simulink model "gm_uz_resolver_multiturn"  (R2025a)
settings: Solver=FixedStepDiscrete  StartTime=0.0  StopTime=2  RelTol=1e-3
settings Model: Creator=jonat  LastModifiedBy=jonat
settings SolverCC: AlgebraicLoopSolver=TrustRegion
settings DataIOCC: LimitDataPoints=on  SaveOutput=off  SaveTime=off
settings OptimizationCC: BlockReduction=off  ConditionallyExecuteInputs=off  DefaultParameterBehavior=Inlined  InheritOutputTypeSmallerThanSingle=on  LifeSpan=inf
settings DebuggingCC: AlgebraicLoopMsg=error  InheritedTsInSrcMsg=none  SingleTaskRateTransMsg=error  UnconnectedInputMsg=warning  UnconnectedOutputMsg=warning  UnconnectedLineMsg=warning  AllowSymbolicDim=off  StrictBusMsg=ErrorOnBusTreatedAsVector  SFUnexpectedBacktrackingDiag=warning  SFNoUnconditionalDefaultTransitionDiag=warning  SFExecutionAtInitializationDiag=none  ArithmeticOperatorsInVariantConditions=warning
settings HardwareCC: ProdBitPerPointer=32.0  ProdBitPerSizeT=32.0  ProdBitPerPtrDiffT=32.0  ProdLargestAtomicFloat=None  ProdIntDivRoundTo=Undefined  ProdEndianess=Unspecified  ProdWordSize=32.0  ProdHWDeviceType=ASIC/FPGA->ASIC/FPGA  ProdEqTarget=off
settings ModelReferenceCC: EnableRefExpFcnMdlSchedulingChecks=on
settings SFSimCC: SimUseLocalCustomCode=off  CustomCodeUndefinedFunction=UseInterfaceOnly
settings RTWCC: RTWUseLocalCustomCode=off  GPUComputeCapability=3.5
settings CodeAppCC: StateflowObjectComments=on
settings GRTTargetCC: TargetLangStandard=C89/C90 (ANSI)
settings ConfigComp: CovScope=ReferencedModels  CovMetricSettings=dw  CovSaveCumulativeToWorkspaceVar=on  CovSaveSingleToWorkspaceVar=on  CovExternalEMLEnable=off  CovSFcnEnable=off

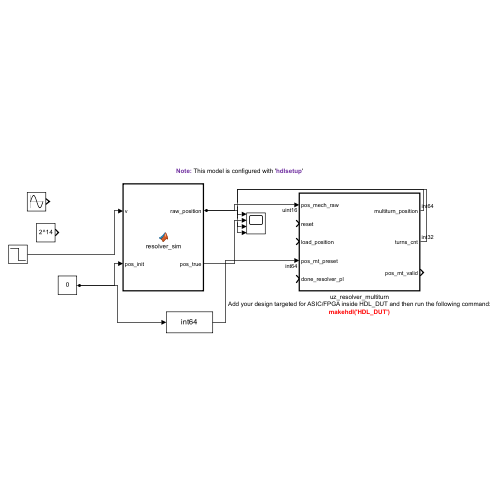
[thumbnail: Simulink's stored preview of the top-level diagram]
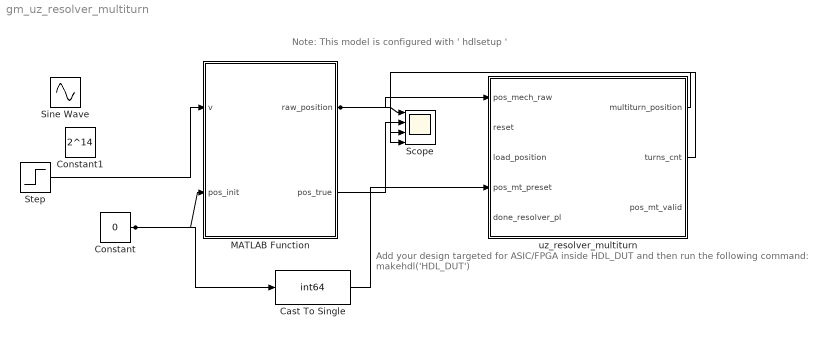
== system gm_uz_resolver_multiturn ==
  note: Add your design targeted for ASIC/FPGA inside HDL_DUT and then run the following command:
      | makehdl('HDL_DUT')
  note: Note: This model is configured with ' hdlsetup '
  Cast To Single : DataTypeConversion  OutDataTypeStr=int64  SaturateOnIntegerOverflow=off  RndMeth=Floor
  Constant : Constant  Value=0
  Constant1 : Constant  Value=2^14
  MATLAB Function : MATLAB Function  TreatAsAtomicUnit=on
  Scope : Scope  NumInputPorts=4
      settings: ActiveDisplayYMinimum=-46082.286781683193  ActiveDisplayYMaximum=89653.10837477204
  Sine Wave : Sin  Amplitude=20000  Frequency=2*pi  SampleTime=0
  Step : Step  Before=2^13  After=-2^13
  uz_resolver_multiturn : Subsystem  TreatAsAtomicUnit=on
  wires:
  uz_resolver_multiturn/2(turns_cnt) -> Scope/4
  Cast To Single/1 -> uz_resolver_multiturn/4(pos_mt_preset)
  uz_resolver_multiturn/1(multiturn_position) -> Scope/3
  MATLAB Function/2(pos_true) -> Scope/2
  MATLAB Function/1(raw_position) -> Scope/1, uz_resolver_multiturn/1(pos_mech_raw)
  Constant/1 -> Cast To Single/1, MATLAB Function/2(pos_init)
  Step/1 -> MATLAB Function/1(v)

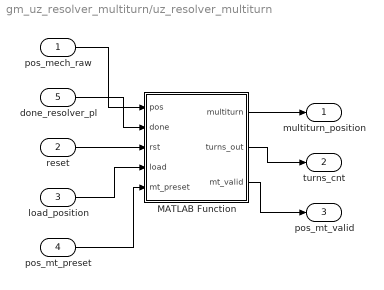
== system gm_uz_resolver_multiturn/uz_resolver_multiturn ==
  pos_mech_raw : Inport  OutDataTypeStr=uint16  PortDimensions=1  SampleTime=0.04
  reset : Inport  Port=2  OutDataTypeStr=boolean  PortDimensions=1  SampleTime=0.04
  load_position : Inport  Port=3  OutDataTypeStr=boolean  PortDimensions=1  SampleTime=0.04
  pos_mt_preset : Inport  Port=4  OutDataTypeStr=fixdt(1, 64, 0)  PortDimensions=1  SampleTime=0.04
  done_resolver_pl : Inport  Port=5  OutDataTypeStr=boolean  PortDimensions=1  SampleTime=0.04
  MATLAB Function : Subsystem
  multiturn_position : Outport  OutDataTypeStr=int64  SampleTime=0.04  VectorParamsAs1DForOutWhenUnconnected=off
  turns_cnt : Outport  Port=2  OutDataTypeStr=int32  SampleTime=0.04
  pos_mt_valid : Outport  Port=3  OutDataTypeStr=boolean  SampleTime=0.04
  wires:
  reset/1 -> MATLAB Function/3(rst)
  pos_mech_raw/1 -> MATLAB Function/1(pos)
  MATLAB Function/3(mt_valid) -> pos_mt_valid/1
  MATLAB Function/1(multiturn) -> multiturn_position/1
  done_resolver_pl/1 -> MATLAB Function/2(done)
  load_position/1 -> MATLAB Function/4(load)
  pos_mt_preset/1 -> MATLAB Function/5(mt_preset)
  MATLAB Function/2(turns_out) -> turns_cnt/1

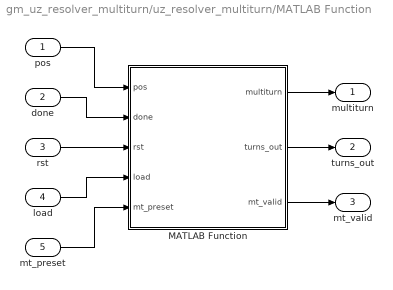
== system gm_uz_resolver_multiturn/uz_resolver_multiturn/MATLAB Function ==
  pos : Inport  OutDataTypeStr=uint16  PortDimensions=1  SampleTime=0.04
  done : Inport  Port=2  OutDataTypeStr=boolean  PortDimensions=1  SampleTime=0.04
  rst : Inport  Port=3  OutDataTypeStr=boolean  PortDimensions=1  SampleTime=0.04
  load : Inport  Port=4  OutDataTypeStr=boolean  PortDimensions=1  SampleTime=0.04
  mt_preset : Inport  Port=5  OutDataTypeStr=fixdt(1, 64, 0)  PortDimensions=1  SampleTime=0.04
  MATLAB Function : MATLAB Function  TreatAsAtomicUnit=on
  multiturn : Outport  SampleTime=0.04
  turns_out : Outport  Port=2  SampleTime=0.04
  mt_valid : Outport  Port=3  SampleTime=0.04
  wires:
  pos/1 -> MATLAB Function/1(pos)
  MATLAB Function/1(multiturn) -> multiturn/1
  done/1 -> MATLAB Function/2(done)
  rst/1 -> MATLAB Function/3(rst)
  load/1 -> MATLAB Function/4(load)
  MATLAB Function/3(mt_valid) -> mt_valid/1
  mt_preset/1 -> MATLAB Function/5(mt_preset)
  MATLAB Function/2(turns_out) -> turns_out/1

== matlab function gm_uz_resolver_multiturn/MATLAB Function ==
  data: v input; raw_position output; pos_init input; pos_true output
function [raw_position, pos_true] = resolver_sim(v, pos_init)
%RESOLVER_SIM  Simuliert einen Resolver als Signalquelle fuer multiturn_counter
%
%   Fuer einen MATLAB Function Block in Simulink (nur Testbench, nicht fuer HDL).
%
%   Eingaenge:
%     v             double   Geschwindigkeit in Counts pro Abtastschritt
%                            (65536 Counts = 1 Umdrehung, |v| < 32768 = 180 Grad)
%     pos_init      double   Startposition in Counts (wird nur im 1. Schritt gelesen)
%
%   Ausgaenge:
%     raw_position  uint16   Singleturn-Rohwert 0 ... 65535 (-> Eingang pos)
%     pos_true      int64    "Wahre" Multiturn-Position in Counts (Referenz)
%
%   Pruefung:
%     multiturn - pos_true muss zwischen zwei rst/load-Ereignissen konstant
%     und ein Vielfaches von 65536 sein. Bei richtig gesetztem mt_preset ist
%     die Differenz 0.

%#codegen

persistent p

if isempty(p)
    p = int64(round(pos_init));
end

% Ausgabe der aktuellen Position
pos_true     = p;
raw_position = uint16(mod(p, int64(65536)));

% Position fuer den naechsten Schritt weiterdrehen
p = p + int64(round(v));

end

== matlab function gm_uz_resolver_multiturn/uz_resolver_multiturn/MATLAB Function/MATLAB Function ==
  settings: fimath=fimath('RoundingMethod', 'Floor','OverflowAction', 'Wrap','ProductMode', 'FullPrecision', 'SumMode', 'FullPrecision')
  data: pos input; done input; multiturn output; rst input; load input; mt_preset input; turns_out output; mt_valid output
function [multiturn, turns_out, mt_valid] = multiturn_counter(pos, done, rst, load, mt_preset)
%MULTITURN_COUNTER  Multiturn-Zaehlung fuer Resolver-Singleturn (uint16)
%
%   Fuer den MATLAB Function Block in Simulink (HDL Coder tauglich).
%   Laeuft im FPGA-Systemtakt (z. B. 100 MHz). Gezaehlt wird nur bei der
%   steigenden Flanke von done (z. B. uz_resolver_pl_interface/done).
%   Funktioniert sowohl, wenn done ein Puls ist, als auch, wenn done ein
%   Pegel ist.
%
%   Eingaenge:
%     pos        uint16   Singleturn-Position (0 ... 65535), z. B. position_raw
%     done       boolean  Neuer, stabiler Positionswert liegt an
%     rst        boolean  Reset: turns = 0, naechster gueltiger Wert wird
%                         ohne Wrap-Pruefung als Startwert uebernommen
%     load       boolean  Letzte bekannte Multiturn-Position uebernehmen
%     mt_preset  int64    Gespeicherte Multiturn-Position (turns*65536 + pos)
%
%   Ausgaenge:
%     multiturn  int64    turns * 65536 + pos_last
%                         (untere 16 Bit = letzter gueltiger Singleturn-Rohwert)
%     turns_out  int32    Umdrehungszaehler
%     mt_valid   boolean  true, sobald multiturn einen gueltigen Bezug hat
%
%   Wrap-Erkennung ueber das Delta zwischen zwei gueltigen Werten:
%     delta < -32768  ->  Ueberlauf vorwaerts  (z. B. 65500 -> 30)
%     delta > +32767  ->  Ueberlauf rueckwaerts (z. B. 30 -> 65500)
%   Voraussetzung: weniger als 180 Grad Drehung zwischen zwei done-Flanken.
%
%   Preset (load):
%     mt_preset wird in turns und pos_last zerlegt. Bei der naechsten
%     done-Flanke laeuft die normale Wrap-Erkennung gegen den neuen Wert.
%     So wird turns korrigiert, wenn die Welle seit dem Speichern ueber die
%     0-Grenze gedreht wurde (Voraussetzung: < 180 Grad seit dem Speichern).
%
%   Prioritaet: rst vor load.
%
%   Die persistenten Variablen werden von HDL Coder als Register umgesetzt.

%#codegen

persistent pos_last turns done_last init_pending

if isempty(pos_last)
    pos_last     = uint16(0);
    turns        = int32(0);
    done_last    = false;
    init_pending = true;
end

% Steigende Flanke von done -> genau ein Takt pro neuem Wert
edge      = done && ~done_last;
done_last = done;

% Reset / Preset
if rst
    turns        = int32(0);
    init_pending = true;                 % naechster gueltiger Wert = Startwert
elseif load
    turns_i64    = bitshift(mt_preset, -16);                    % floor
    turns        = int32(turns_i64);
    pos_last     = uint16(mt_preset - bitshift(turns_i64, 16)); % 0 ... 65535
    init_pending = false;
end

% Zaehlung nur bei neuem, gueltigem Wert
if edge
    if init_pending
        pos_last     = pos;              % Startwert ohne Wrap-Pruefung
        init_pending = false;
    else
        % Delta in int32 bilden (MATLAB-Integer saettigen, kein int16-Cast)
        delta = int32(pos) - int32(pos_last);
        if delta < int32(-32768)
            turns = turns + int32(1);
        elseif delta > int32(32767)
            turns = turns - int32(1);
        end
        pos_last = pos;
    end
end

% Ausgabe: {turns, pos_last}
multiturn = bitshift(int64(turns), 16) + int64(pos_last);
turns_out = turns;
mt_valid  = ~init_pending;

end
